simulink model "AvonGasTurbineDgTwin_fixed"  (R2024b)
settings: Solver=VariableStepAuto  StartTime=0  StopTime=7200  FixedStep=1  RelTol=1e-3  EnableMultiTasking=on
InitFcn:
  | warning off
model workspace (MAT data in the model file):
  FAULT_01_AirIntakeFilterFouling_enable = 1
  FAULT_02_CompBladeFouling_enable = 1
  FAULT_03_CompBladeDamage_enable = 1
  FAULT_04_CompSurgeStall_enable = 1
  FAULT_05_DiffuserDamage_enable = 1
  FAULT_06_IGVStuck_enable = 1
  FAULT_07_FuelPrssRegulatorStuck_enable = 1
  FAULT_08_FuelValveLeakage_enable = 1
  FAULT_09_FuelContamination_enable = 1
  FAULT_10_FuelLineBlockage_enable = 1
  FAULT_11_FuelPumpDegradation_enable = 1
  FAULT_12_FuelSupplyPressDrop_enable = 1
  FAULT_13_FGSupplyPressOscillation_enable = 1
  FAULT_14_FGValvePartialOpening_enable = 1
  FAULT_15_FGValveActuatorDelay_enable = 1
  FAULT_15_FuelPressReg_enable = 0
  FAULT_16_CombLinerDamage_enable = 1
  FAULT_16_FuelValveLeak_enable = 0
  FAULT_17_FuelNozzleClogging_enable = 1
  FAULT_18_CombustionFlameOscillation_enable = 1
  FAULT_19_CombustionInstability_enable = 1
  FAULT_20_HotGasPathTempIncrease_enable = 1
  FAULT_21_GGTurbFouling_enable = 1
  FAULT_22_GGTurbBladeDamage_enable = 1
  FAULT_23_GGNozzleBlockage_enable = 1
  FAULT_24_GGSealDegradation_enable = 1
  FAULT_25_GGInletPressureLoss_enable = 1
  FAULT_26_PTFouling_enable = 1
  FAULT_27_PTBladeDamage_enable = 1
  FAULT_28_PTNozzleDamage_enable = 1
  FAULT_29_PTSealDegradation_enable = 1
  FAULT_30_PTBearingWear_enable = 1
  FAULT_31_PTPowerLoss_enable = 1
  FAULT_32_PTStackBlockage_enable = 1
  FAULT_33_SensorEnhancement_enable = 1
  FAULT_34_SensorDegradation_enable = 1
  FAULT_35_SensorEnhanceStep_enable = 1
  FAULT_36_SensorDegradeStep_enable = 1
  FAULT_37_SensorFreez_enable = 1
  FAULT_38_GGSpeedSensor_enable = 1
  FAULT_39_PTSpeedSensor_enable = 1
  FAULT_40_FGSensorOffset_enable = 1
  FAULT_41_FGSensorDrift_enable = 1
  FAULT_42_ControlLoopOscillation_enable = 1
  GOV_GG_BASELINE = 10
  GOV_GG_DROOP_PCT = 0.04
  GOV_PT_BASELINE = 10
  GOV_PT_DROOP_PCT = 0.04
  SW_Manual_Switch1_enable = 1
  SW_Manual_Switch2_enable = 1
  SW_Manual_Switch3_enable = 1
  SW_Manual_Switch4_enable = 1
  SW_Manual_Switch_enable = 1
undefined symbols (not defined in the file or in its folder): ENV_ambient_moisture_pct, ENV_comp_inlet_press_kPa, ENV_FG_pressure_kPa, ENV_FG_temp_C, SP_POWER_CMD
libraries: slpidlib x3, simulink x2
(part 4 of 4)

== system AvonGasTurbineDgTwin_fixed/Subsystem/Combustor1/combustion chamber 1/Cp fuel ==
  Tinlet : Inport
  Cp : Fcn  Expr=(1.702+9.081*1e-3*u(1)-2.164*1e-6*u(1)^2)*0.5183  SampleTime=1
  oC-----> K : Fcn  Expr=(u(1)+273.15)  SampleTime=1
  Cp(T) : Outport
  wires:
  oC-----> K/1 -> Cp/1
  Cp/1 -> Cp(T)/1
  Tinlet/1 -> oC-----> K/1

== system AvonGasTurbineDgTwin_fixed/Subsystem/FG MCV model1/CV model chamber 2/Cp FG ==
  Tinlet : Inport
  Cp : Fcn  Expr=(1.702+9.081*1e-3*u(1)-2.164*1e-6*u(1)^2)*0.5183  SampleTime=1
  oC-----> K : Fcn  Expr=(u(1)+273.15)  SampleTime=1
  Cp(T) : Outport
  wires:
  oC-----> K/1 -> Cp/1
  Cp/1 -> Cp(T)/1
  Tinlet/1 -> oC-----> K/1

== system AvonGasTurbineDgTwin_fixed/Subsystem/FG MCV model1/CV model chamber 2/density FG ==
  FG_prss : Inport
  FG_temp : Inport  Port=2
  1+0.257*Pr-0.533*Pr/Tr : Fcn  Expr=1+0.257*u(1)-0.533*u(1)/u(2)
  Constant3 : Constant  Value=273.15
  Mux : Mux  Inputs=2
  Sum2 : Sum  Inputs=|++
  Tcr : Constant  Value=191
  Tnormal : Constant  Value=273.15+15
  Tnormal/T : Product  Inputs=*/  RndMeth=Zero
  Zn : Constant  Value=0.9974
  density @ n.c.1 : Gain  Gain=0.78862
  density @ n.c.2 : Gain  Gain=1/14.89
  p/pcr : Product  Inputs=*/  RndMeth=Zero
  p/pnormal1 : Product  Inputs=/*  RndMeth=Zero
  p1 : Product  Inputs=3  RndMeth=Zero
  pcr : Constant  Value=4640
  pnormal2 : Constant  Value=101.3
  t/Tc : Product  Inputs=*/  RndMeth=Zero
  z correction : Product  Inputs=/*  RndMeth=Zero
  density : Outport
  wires:
  Tnormal/1 -> Tnormal/T/1
  Constant3/1 -> Sum2/2
  Sum2/1 -> Tnormal/T/2, t/Tc/1
  pcr/1 -> p/pcr/2
  Tcr/1 -> t/Tc/2
  Zn/1 -> z correction/2
  FG_temp/1 -> Sum2/1
  p/pcr/1 -> Mux/1  "pr"
  t/Tc/1 -> Mux/2  "Tr"
  density @ n.c.2/1 -> density/1
  z correction/1 -> p1/3
  Mux/1 -> 1+0.257*Pr-0.533*Pr/Tr/1
  1+0.257*Pr-0.533*Pr/Tr/1 -> z correction/1
  FG_prss/1 -> p/pnormal1/2, p/pcr/1
  pnormal2/1 -> p/pnormal1/1
  p/pnormal1/1 -> p1/2
  p1/1 -> density @ n.c.1/1
  density @ n.c.1/1 -> density @ n.c.2/1
  Tnormal/T/1 -> p1/1

== system AvonGasTurbineDgTwin_fixed/Subsystem/FG MCV model1/Subsystem1/Z ==
  T : Inport
  P : Inport  Port=2
  1+0.257*Pr-0.533*Pr/Tr1 : Fcn  Expr=1+0.257*u(1)-0.533*u(1)/u(2)
  Mux5 : Mux  Inputs=2
  Tcr1 : Constant  Value=191
  p/pcr1 : Product  Inputs=*/  RndMeth=Zero
  pcr1 : Constant  Value=4640
  t/Tc1 : Product  Inputs=*/  RndMeth=Zero
  Z : Outport
  wires:
  Mux5/1 -> 1+0.257*Pr-0.533*Pr/Tr1/1
  P/1 -> p/pcr1/1
  T/1 -> t/Tc1/1
  Tcr1/1 -> t/Tc1/2
  1+0.257*Pr-0.533*Pr/Tr1/1 -> Z/1
  t/Tc1/1 -> Mux5/2  "Tr"
  pcr1/1 -> p/pcr1/2
  p/pcr1/1 -> Mux5/1  "pr"

== system AvonGasTurbineDgTwin_fixed/Subsystem/GasGenerator/Turbine section/FAULT_21_GGTurbFouling ==
  In1 : Inport
  FAULT_21_multiplier : FromWorkspace  VariableName=FAULT_21_multiplier  SampleTime=-1
  Mux : Mux  Inputs=2
  Product : Product
  Scope{,1..3} (4 alike) : Scope  Commented=on
  Out1 : Outport
  wires:
  FAULT_21_multiplier/1 -> Product/1, Scope/1
  In1/1 -> Scope1/1, Mux/2, Product/2
  Product/1 -> Mux/1, Scope2/1, Out1/1
  Mux/1 -> Scope3/1

== system AvonGasTurbineDgTwin_fixed/Subsystem/GasGenerator/Turbine section/FAULT_22_GGTurbBladeDamage ==
  In1 : Inport
  FAULT_22_multiplier : FromWorkspace  VariableName=FAULT_22_multiplier  SampleTime=-1
  Mux : Mux  Inputs=2
  Product : Product
  Scope{,1..3} (4 alike) : Scope  Commented=on
  Out1 : Outport
  wires:
  FAULT_22_multiplier/1 -> Product/1, Scope/1
  In1/1 -> Scope1/1, Mux/2, Product/2
  Product/1 -> Mux/1, Scope2/1, Out1/1
  Mux/1 -> Scope3/1

== system AvonGasTurbineDgTwin_fixed/Subsystem/GasGenerator/Turbine section/hot_air ==
  Tinlet : Inport
  Cp(T) : Fcn  Expr=(3.355+5.75*1e-4*u(1)-1600*u(1)^(-2))*0.28714  SampleTime=1
  Cp(P1,T1) : Outport
  wires:
  Cp(T)/1 -> Cp(P1,T1)/1
  Tinlet/1 -> Cp(T)/1

== system AvonGasTurbineDgTwin_fixed/Subsystem/GasGenerator/cooling 1/Cp Temp ==
  Tinlet : Inport
  Cp : Fcn  Expr=(3.355+5.75*1e-4*u(1)-1600*u(1)^(-2))*0.28714  SampleTime=1
  Cp(T) : Outport
  wires:
  Cp/1 -> Cp(T)/1
  Tinlet/1 -> Cp/1  "Kelvin"

== system AvonGasTurbineDgTwin_fixed/Subsystem/GasGenerator/cooling 1/Cp Temp air ==
  Tinlet : Inport
  Cp : Fcn  Expr=(3.355+5.75*1e-4*u(1)-1600*u(1)^(-2))*0.28714  SampleTime=1
  Cp(T) : Outport
  wires:
  Tinlet/1 -> Cp/1  "Kelvin"
  Cp/1 -> Cp(T)/1

== system AvonGasTurbineDgTwin_fixed/Subsystem/GasGenerator/cooling 1/Cp Temp hot gas ==
  Tinlet : Inport
  Cp : Fcn  Expr=(3.355+5.75*1e-4*u(1)-1600*u(1)^(-2))*0.28714  SampleTime=1
  Cp(T) : Outport
  wires:
  Cp/1 -> Cp(T)/1
  Tinlet/1 -> Cp/1  "Kelvin"

== system AvonGasTurbineDgTwin_fixed/Subsystem/GasGenerator/cooling 2/Cp Temp ==
  Tinlet : Inport
  Cp : Fcn  Expr=(3.355+5.75*1e-4*u(1)-1600*u(1)^(-2))*0.28714  SampleTime=1
  Cp(T) : Outport
  wires:
  Tinlet/1 -> Cp/1  "Kelvin"
  Cp/1 -> Cp(T)/1

== system AvonGasTurbineDgTwin_fixed/Subsystem/GasGenerator/cooling 2/Cp Temp air ==
  Tinlet : Inport
  Cp : Fcn  Expr=(3.355+5.75*1e-4*u(1)-1600*u(1)^(-2))*0.28714  SampleTime=1
  Cp(T) : Outport
  wires:
  Cp/1 -> Cp(T)/1
  Tinlet/1 -> Cp/1  "Kelvin"

== system AvonGasTurbineDgTwin_fixed/Subsystem/GasGenerator/cooling 2/Cp Temp hot gas ==
  Tinlet : Inport
  Cp : Fcn  Expr=(3.355+5.75*1e-4*u(1)-1600*u(1)^(-2))*0.28714  SampleTime=1
  Cp(T) : Outport
  wires:
  Tinlet/1 -> Cp/1  "Kelvin"
  Cp/1 -> Cp(T)/1

== system AvonGasTurbineDgTwin_fixed/Subsystem/PowerTurbine/Turbine section/FAULT_26_PTFouling ==
  In1 : Inport
  FAULT_26_multiplier : FromWorkspace  VariableName=FAULT_26_multiplier  SampleTime=-1
  Mux : Mux  Inputs=2
  Product : Product
  Scope{,1..3} (4 alike) : Scope  Commented=on
  Out1 : Outport
  wires:
  FAULT_26_multiplier/1 -> Product/1, Scope/1
  In1/1 -> Scope1/1, Mux/2, Product/2
  Product/1 -> Mux/1, Scope2/1, Out1/1
  Mux/1 -> Scope3/1

== system AvonGasTurbineDgTwin_fixed/Subsystem/PowerTurbine/Turbine section/FAULT_27_PTBladeDamage ==
  In1 : Inport
  FAULT_27_multiplier : FromWorkspace  VariableName=FAULT_27_multiplier  SampleTime=-1
  Mux : Mux  Inputs=2
  Product : Product
  Scope{,1..3} (4 alike) : Scope  Commented=on
  Out1 : Outport
  wires:
  FAULT_27_multiplier/1 -> Product/1, Scope/1
  In1/1 -> Scope1/1, Mux/2, Product/2
  Product/1 -> Mux/1, Scope2/1, Out1/1
  Mux/1 -> Scope3/1

== system AvonGasTurbineDgTwin_fixed/Subsystem/PowerTurbine/Turbine section/FAULT_32_PTStackBlockage ==
  In1 : Inport
  FAULT_32_multiplier : FromWorkspace  VariableName=FAULT_32_multiplier  SampleTime=-1
  Mux : Mux  Inputs=2
  Product : Product
  Scope{,1..3} (4 alike) : Scope  Commented=on
  Out1 : Outport
  wires:
  FAULT_32_multiplier/1 -> Product/1, Scope/1
  In1/1 -> Scope1/1, Mux/2, Product/2
  Product/1 -> Mux/1, Scope2/1, Out1/1
  Mux/1 -> Scope3/1

== system AvonGasTurbineDgTwin_fixed/Subsystem/PowerTurbine/Turbine section/hot_air ==
  Tinlet : Inport
  Cp(T) : Fcn  Expr=(3.355+5.75*1e-4*u(1)-1600*u(1)^(-2))*0.28714  SampleTime=1
  Cp(P1,T1) : Outport
  wires:
  Tinlet/1 -> Cp(T)/1
  Cp(T)/1 -> Cp(P1,T1)/1

== system AvonGasTurbineDgTwin_fixed/Subsystem/PowerTurbine/rotor dynamic/FAULT_30_PTBearingWear ==
  In1 : Inport
  FAULT_30_multiplier : FromWorkspace  VariableName=FAULT_30_multiplier  SampleTime=-1
  Mux : Mux  Inputs=2
  Product : Product
  Scope{,1..3} (4 alike) : Scope  Commented=on
  Out1 : Outport
  wires:
  FAULT_30_multiplier/1 -> Product/1, Scope/1
  In1/1 -> Scope1/1, Mux/2, Product/2
  Product/1 -> Mux/1, Scope2/1, Out1/1
  Mux/1 -> Scope3/1

== system AvonGasTurbineDgTwin_fixed/Subsystem/comp_temp1/Cp_com_in/Cp dry air ==
  Tinlet : Inport
  Cp : Fcn  Expr=(3.355+5.75*1e-4*u(1)-1600*u(1)^(-2))*0.28714  SampleTime=1
  Cp(T) : Outport
  wires:
  Cp/1 -> Cp(T)/1
  Tinlet/1 -> Cp/1

== system AvonGasTurbineDgTwin_fixed/Subsystem/comp_temp1/Cp_com_in/Cp steam ==
  Tinlet : Inport
  Cp : Fcn  Expr=(3.47+1.45*1e-3*u(1)+1.21*1e4*u(1)^(-2))*0.4615  SampleTime=1
  Cp(T) : Outport
  wires:
  Tinlet/1 -> Cp/1
  Cp/1 -> Cp(T)/1

== system AvonGasTurbineDgTwin_fixed/Subsystem/comp_temp1/Cp_com_in/Specific humidity ==
  humidity : Inport
  Press_kPa : Inport  Port=2
  temp : Inport  Port=3
  1/100 : Gain  Gain=0.01
  Ps (saturation pressure) : Fcn  Expr=((u-200.5754)/81.4934)^6.1556  SampleTime=1
  Scope11 : Scope
  "Specific humidity " : Gain  Gain=0.6219
  Sum : Sum  Inputs=-+
  x : Product  RndMeth=Zero
  x1 : Product  Inputs=*/  RndMeth=Zero
  y : Outport
  wires:
  Ps (saturation pressure)/1 -> Scope11/1, x/1
  "Specific humidity "/1 -> y/1
  x1/1 -> "Specific humidity "/1
  Sum/1 -> x1/2
  Press_kPa/1 -> Sum/2
  x/1 -> x1/1, Sum/1  "pv"
  1/100/1 -> x/2
  humidity/1 -> 1/100/1
  temp/1 -> Ps (saturation pressure)/1
